simulink model "CTV_GMEKF_Simulation"  (R2026a)
settings: Solver=VariableStepAuto
undefined symbols (not defined in the file or in its folder): barometer_st, gps_st, imu_st, lidar_frames, qc
settings Model: DataDictionary=NavigationDictionary.sldd  Creator=David  LastModifiedBy=David

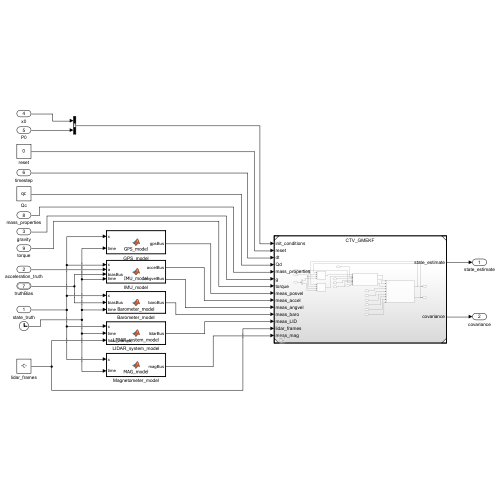
[thumbnail: Simulink's stored preview of the top-level diagram]
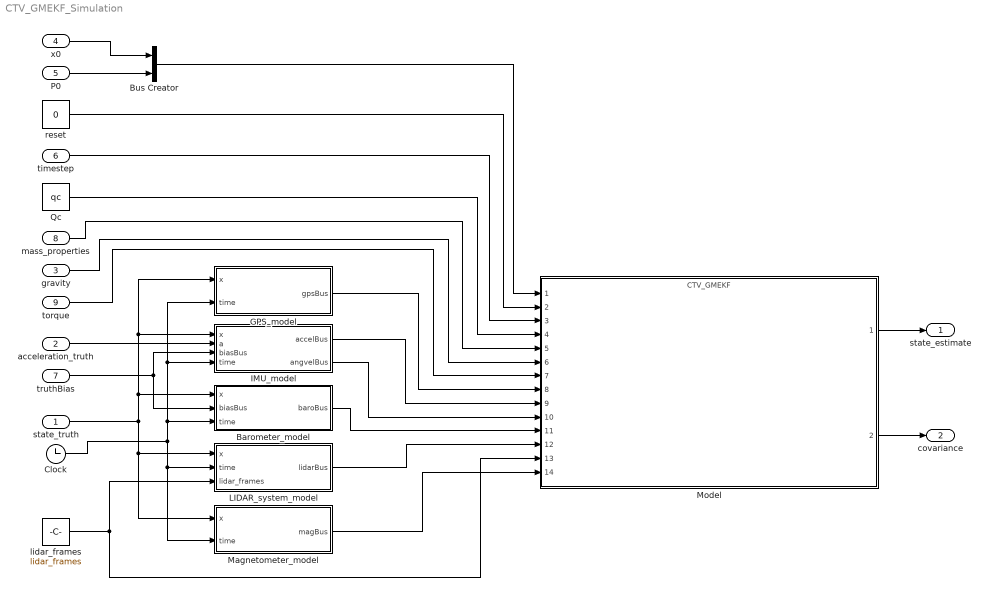
== system CTV_GMEKF_Simulation ==
  state_truth : Inport
  acceleration_truth : Inport  Port=2
  gravity : Inport  Port=3
  x0 : Inport  Port=4
  P0 : Inport  Port=5
  timestep : Inport  Port=6
  truthBias : Inport  Port=7  OutDataTypeStr=Bus: biasBus
  mass_properties : Inport  Port=8
  torque : Inport  Port=9
  Barometer_model : MATLAB Function  TreatAsAtomicUnit=on  SystemSampleTime=barometer_st
  Bus Creator : BusCreator  Inputs=2  OutDataTypeStr=Bus: InitConditions
  Clock : Clock
  GPS_model : MATLAB Function  TreatAsAtomicUnit=on  SystemSampleTime=gps_st
  IMU_model : MATLAB Function  TreatAsAtomicUnit=on  SystemSampleTime=imu_st
  LIDAR_system_model : MATLAB Function  TreatAsAtomicUnit=on
  Magnetometer_model : MATLAB Function  TreatAsAtomicUnit=on
  Model : ModelReference  ModelNameDialog=CTV_GMEKF.slx  SimulationMode=Normal  ModelReferenceVersion=1.38
  Qc : Constant  Value=qc  OutDataTypeStr=ValueType: Qc
  lidar_frames : Constant  Value=lidar_frames  OutDataTypeStr=Bus: lidarFrameBus
  reset : Constant  Value=0
  state_estimate : Outport  PortDimensions=[20 1]
  covariance : Outport  Port=2  PortDimensions=[19 19]
  wires:
  Model/1 -> state_estimate/1
  Model/2 -> covariance/1
  state_truth/1 -> Magnetometer_model/1(x), LIDAR_system_model/1(x), Barometer_model/1(x), GPS_model/1(x), IMU_model/1(x)
  acceleration_truth/1 -> IMU_model/2(a)
  Clock/1 -> Magnetometer_model/2(time), LIDAR_system_model/2(time), IMU_model/4(time), GPS_model/2(time), Barometer_model/3(time)
  P0/1 -> Bus Creator/2
  x0/1 -> Bus Creator/1
  Bus Creator/1 -> Model/1
  truthBias/1 -> Barometer_model/2(biasBus), IMU_model/3(biasBus)
  reset/1 -> Model/2
  timestep/1 -> Model/3
  lidar_frames/1 -> Model/13, LIDAR_system_model/3(lidar_frames)
  torque/1 -> Model/7
  gravity/1 -> Model/6
  mass_properties/1 -> Model/5
  Qc/1 -> Model/4
  GPS_model/1(gpsBus) -> Model/8
  IMU_model/1(accelBus) -> Model/9
  IMU_model/2(angvelBus) -> Model/10
  Magnetometer_model/1(magBus) -> Model/14
  Barometer_model/1(baroBus) -> Model/11
  LIDAR_system_model/1(lidarBus) -> Model/12

== matlab function CTV_GMEKF_Simulation/IMU_model ==
  data: x input; accelBus output; angvelBus output; a input; biasBus input; time input
function [accelBus, angvelBus] = IMU_model(x, a, biasBus, time)
ab = biasBus.accelBias;
gb = biasBus.accelBias;
[accelBus, angvelBus] = imu_model(x, a, ab, gb, time);
end

== matlab function CTV_GMEKF_Simulation/GPS_model ==
  data: x input; gpsBus output; time input
function gpsBus = GPS_model(x, time)
gpsBus = gps_model(x, time);
end

== matlab function CTV_GMEKF_Simulation/Barometer_model ==
  data: x input; biasBus input; baroBus output; time input
function baroBus = Barometer_model(x, biasBus, time)
bb = biasBus.baroBias;
baroBus = barometer_model(x, bb, time);
end

== matlab function CTV_GMEKF_Simulation/LIDAR_system_model ==
  data: x input; lidarBus output; time input; lidar_frames input
function lidarBus = LIDAR_system_model(x, time, lidar_frames)
lidarBus = lidar_system_model(x, time, lidar_frames);
end

== matlab function CTV_GMEKF_Simulation/Magnetometer_model ==
  data: x input; magBus output; time input
function magBus = MAG_model(x, time)
magBus = mag_model(x, time);
end
